simulink model "DINAMICA_SIMULINK"  (R2023b)
settings: Solver=ode4  StartTime=0.0  StopTime=24  FixedStep=0.001  RelTol=1e-3
settings Model: Creator=mondr  LastModifiedBy=mondr

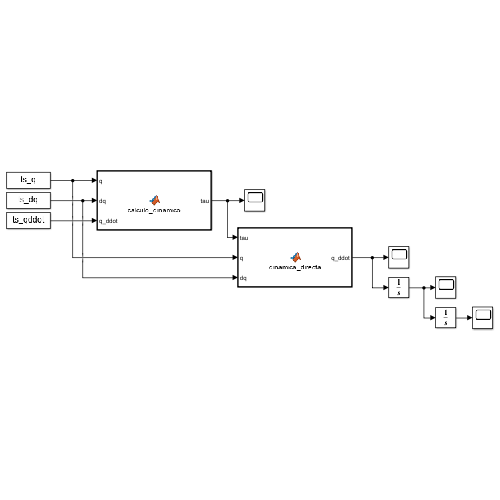
[thumbnail: Simulink's stored preview of the top-level diagram]
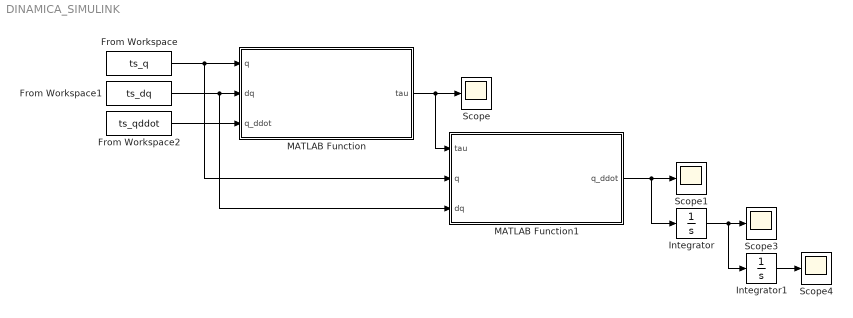
== system DINAMICA_SIMULINK ==
  From Workspace : FromWorkspace  VariableName=ts_q
  From Workspace1 : FromWorkspace  VariableName=ts_dq
  From Workspace2 : FromWorkspace  VariableName=ts_qddot
  Integrator : Integrator
  Integrator1 : Integrator  InitialCondition=[0; -pi/2; pi/2]
  MATLAB Function : MATLAB Function  TreatAsAtomicUnit=on
  MATLAB Function1 : MATLAB Function  TreatAsAtomicUnit=on
  Scope{,1,3..4} (4 alike) : Scope
  wires:
  From Workspace/1 -> MATLAB Function1/2(q), MATLAB Function/1(q)
  From Workspace1/1 -> MATLAB Function1/3(dq), MATLAB Function/2(dq)
  From Workspace2/1 -> MATLAB Function/3(q_ddot)
  MATLAB Function/1(tau) -> MATLAB Function1/1(tau), Scope/1
  MATLAB Function1/1(q_ddot) -> Integrator/1, Scope1/1
  Integrator/1 -> Integrator1/1, Scope3/1
  Integrator1/1 -> Scope4/1

== matlab function DINAMICA_SIMULINK/MATLAB Function ==
  data: q input; tau output; dq input; q_ddot input
function tau = calculo_dinamico(q, dq, q_ddot)

    M = M_func(q(2), q(3));
    C = C_func(q(2), q(3), dq(1), dq(2), dq(3));
    g = gq_func(q(2), q(3));
   
    tau = M * q_ddot + C * dq + g;
    
end

== matlab function DINAMICA_SIMULINK/MATLAB Function1 ==
  data: tau input; q input; q_ddot output; dq input
function q_ddot = dinamica_directa(tau, q, dq)

    M = M_func(q(2), q(3));
    C = C_func(q(2), q(3), dq(1), dq(2), dq(3));
    g = gq_func(q(2), q(3));
    
    q_ddot = M \ (tau - C*dq - g);
    
end
